simulink model "kinematics_model"  (R2024a)
settings: Solver=VariableStepAuto  StartTime=0.0  StopTime=10.0  RelTol=1e-3
undefined symbols (not defined in the file): dh_table
settings Model: Creator=Milon  LastModifiedBy=Milon

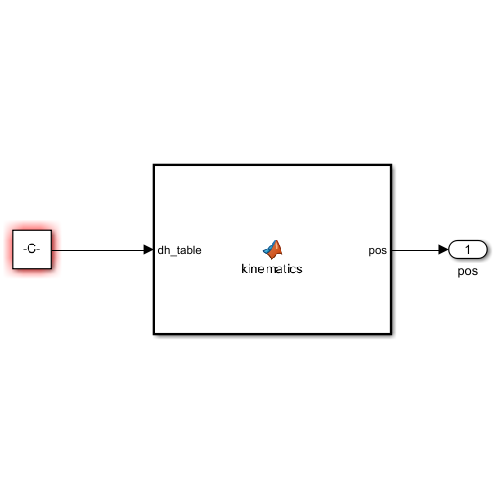
[thumbnail: Simulink's stored preview of the top-level diagram]
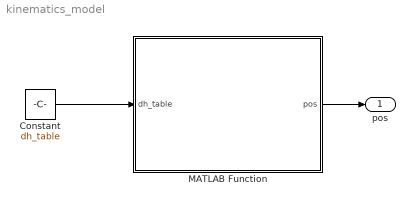
== system kinematics_model ==
  Constant : Constant  Value=dh_table
  MATLAB Function : MATLAB Function  TreatAsAtomicUnit=on
  pos : Outport
  wires:
  MATLAB Function/1(pos) -> pos/1
  Constant/1 -> MATLAB Function/1(dh_table)

== matlab function kinematics_model/MATLAB Function ==
  data: dh_table input; pos output
function pos = kinematics(dh_table)

    t1 = dh_table(1, 1);
    t2 = dh_table(2, 1);
    t3 = dh_table(3, 1);
    
    L1 = dh_table(1, 3);
    L2 = dh_table(2, 3);
    L3 = dh_table(3, 3);


    phi = t1 + t2 + t3;
    x = L1 * cos(t1) + L2 * cos(t1 + t2) + L3 * cos(phi);
    y = L1 * sin(t1) + L2 * sin(t1 + t2) + L3 * sin(phi);

    pos = [x, y, phi];
end
